simulink model "mcb_pmsm_foc_sensorless_f28069MLaunchPad"  (R2024a)
settings: Solver=FixedStepDiscrete  StartTime=0.0  StopTime=8  RelTol=1e-3  EnableMultiTasking=on
InitFcn:
  | mcb_pmsm_foc_sensorless_f28069MLaunchPad_datascript;
undefined symbols (not defined in the file): acceleration, Down, GPTRIP1SEL, GPTRIP2SEL, inverter, MAX_OL_NEG_SPD, MAX_OL_POS_SPD, MAX_OL_VD_LIMIT, MIN_CL_NEG_SPD, MIN_CL_POS_SPD, MIN_OL_VD_LIMIT, one_sec_tick, PI_params, pmsm, PU_System, RAMP_STEP_SIZE, target, Ts, Ts_motor, Ts_simulink, Ts_speed, two_sec_tick, TZ1, TZ2, Up
libraries: mcbcontrolslib x16, c2802xlib x5, simulink x4, c280xlib x4, slpidlib x3, mcbpositiondecoderlib x3, c2806xlib x3, mcbsensorlessestimatorlib x2, svdschedulerlib x2, mcbplantlib x1, autolibpmsmexterior x1
(part 1 of 3)
settings Model: ExtModeTrigDuration=8  Creator=The MathWorks, Inc.  LastModifiedBy=hirah
settings SolverCC: AlgebraicLoopSolver=TrustRegion  AutoInsertRateTranBlk=on
settings DataIOCC: LimitDataPoints=on  SaveFormat=Array  SaveOutput=off  SaveTime=off  ReturnWorkspaceOutputs=off
settings OptimizationCC: DefaultParameterBehavior=Inlined  DefaultUnderspecifiedDataType=single  OptimizeBlockIOStorage=off  BufferReuse=off  GlobalBufferReuse=off  ExpressionFolding=off  ExpressionDepthLimit=2147483647  LocalBlockOutputs=off  InitFltsAndDblsToZero=on  NoFixptDivByZeroProtection=on  EfficientFloat2IntCast=on  EfficientMapNaN2IntZero=off  LifeSpan=inf  MaxStackSize=1024  OptimizeDataStoreBuffers=off  BusAssignmentInplaceUpdate=off  DenormalBehavior=FlushToZero  EfficientTunableParamExpr=on
settings DebuggingCC: AlgebraicLoopMsg=error  ArtificialAlgebraicLoopMsg=error  CheckSSInitialOutputMsg=off  MergeDetectMultiDrivingBlocksExec=none  SolverPrmCheckMsg=warning  InheritedTsInSrcMsg=none  MultiTaskDSMMsg=none  MultiTaskCondExecSysMsg=none  TasksWithSamePriorityMsg=none  SigSpecEnsureSampleTimeMsg=none  ParameterPrecisionLossMsg=none  ParameterTunabilityLossMsg=error  FcnCallInpInsideContextMsg=warning  UnconnectedInputMsg=warning  UnconnectedOutputMsg=warning  UnconnectedLineMsg=warning  AllowSymbolicDim=off  StateNameClashWarn=warning  SFUnexpectedBacktrackingDiag=warning  SFNoUnconditionalDefaultTransitionDiag=warning  SFExecutionAtInitializationDiag=none  ArithmeticOperatorsInVariantConditions=warning
settings HardwareCC: ProdBitPerChar=16  ProdBitPerInt=16  ProdBitPerPointer=32  ProdBitPerSizeT=32  ProdBitPerPtrDiffT=32  ProdLargestAtomicInteger=Integer  ProdLargestAtomicFloat=None  ProdWordSize=16  ProdLongLongMode=on  ProdHWDeviceType=Texas Instruments->C2000  TargetBitPerChar=16  TargetBitPerInt=16  TargetBitPerPointer=16  TargetLargestAtomicInteger=Integer  TargetIntDivRoundTo=Zero  TargetEndianess=LittleEndian  TargetWordSize=16  TargetHWDeviceType=Texas Instruments->C2000
settings ModelReferenceCC: EnableRefExpFcnMdlSchedulingChecks=on  PropagateSignalLabelsOutOfModel=off
settings SFSimCC: SimUseLocalCustomCode=off  MATLABDynamicMemAlloc=off
settings RTWCC: Description=Embedded Coder  SystemTargetFile=ert.tlc  HardwareBoard=TI Piccolo F28069M LaunchPad  TemplateMakefile=ert_default_tmf  PostCodeGenCommand=; codertarget.postCodeGenHookCommand(h)  GenerateReport=on  RTWUseLocalCustomCode=off  Toolchain=Texas Instruments Code Composer Studio (C2000)  BuildConfiguration=Faster Runs  IncludeHyperlinkInReport=on  LaunchReport=on  GenerateTraceInfo=on  GenerateTraceReport=on  GenerateTraceReportSl=on  GenerateTraceReportSf=on  GenerateTraceReportEml=on  GPUComputeCapability=3.5  DLArmComputeVersion=19.05
settings CodeAppCC: IgnoreCustomStorageClasses=off  CustomSymbolStrType=$N$R$M  StateflowObjectComments=on  InternalIdentifier=Classic
settings ERTTargetCC: TargetFcnLib=ansi_tfl_tmw_new.mat  CodeReplacementLibrary=TI C28x  MultiwordLength=2048  ParMdlRefBuildCompliant=off  CompOptLevelCompliant=off  ConcurrentExecutionCompliant=off  CPPClassGenCompliant=off  ExtModeStaticAllocSize=2000  ExtModeMexFile=TIC2000ExternalModeOpen  ExtModeIntrfLevel=Level2 - Open  ConvertIfToSwitch=off  SuppressUnreachableDefaultCases=off  MemSecPackage=tic2000demospkg
settings ConfigComp: CovMetricSettings=dw  CovSaveCumulativeToWorkspaceVar=on  CovSaveSingleToWorkspaceVar=on  CovExternalEMLEnable=off  CovSFcnEnable=off

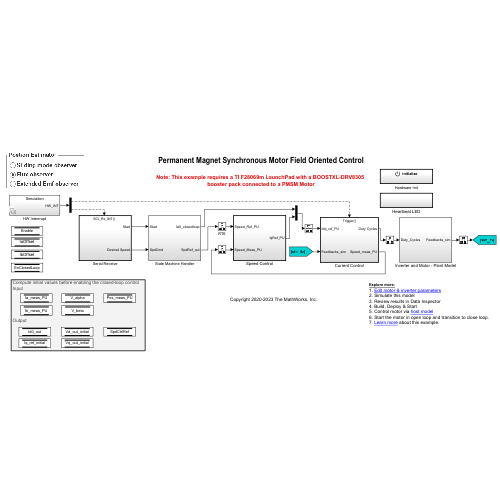
[thumbnail: Simulink's stored preview of the top-level diagram]
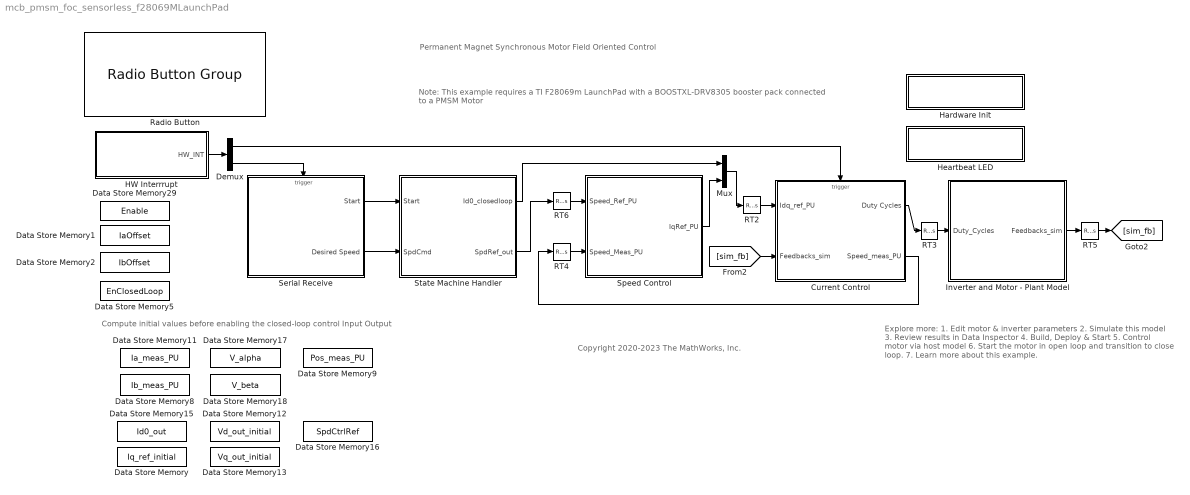
== system mcb_pmsm_foc_sensorless_f28069MLaunchPad ==
  note: Permanent Magnet Synchronous Motor Field Oriented Control
  note: Copyright 2020-2023 The MathWorks, Inc.
  note: Note: This example requires a TI F28069m LaunchPad with a BOOSTXL-DRV8305
      | booster pack connected to a PMSM Motor
  note: Explore more:
      | 1. Edit motor & inverter parameters
      | 2. Simulate this model
      | 3. Review results in Data Inspector
      | 4. Build, Deploy & Start
      | 5. Control motor via host model
      | 6. Start the motor in open loop and transition to close loop.
      | 7. Learn more about this example.
  note: Compute initial values before enabling the closed-loop control
      | Input
      |
      |
      |
      |
      |
      | Output
  Current Control : Subsystem
      settings: RTWSystemCode=Nonreusable function
  Data Store Memory : DataStoreMemory  DataStoreName=Iq_ref_initial  WriteAfterWriteMsg=warning  ShowAdditionalParam=off  OutDataTypeStr=dataType
  Data Store Memory1 : DataStoreMemory  DataStoreName=IaOffset  InitialValue=inverter.CtSensAOffset  ShowAdditionalParam=off
  Data Store Memory11 : DataStoreMemory  DataStoreName=Ia_meas_PU  WriteAfterWriteMsg=warning  ShowAdditionalParam=off  OutDataTypeStr=dataType
  Data Store Memory12 : DataStoreMemory  DataStoreName=Vd_out_initial  WriteAfterWriteMsg=warning  ShowAdditionalParam=off  OutDataTypeStr=dataType
  Data Store Memory13 : DataStoreMemory  DataStoreName=Vq_out_initial  WriteAfterWriteMsg=warning  ShowAdditionalParam=off  OutDataTypeStr=dataType
  Data Store Memory15 : DataStoreMemory  DataStoreName=Id0_out  InitialValue=0.1  ShowAdditionalParam=off  OutDataTypeStr=dataType
  Data Store Memory16 : DataStoreMemory  DataStoreName=SpdCtrlRef  InitialValue=0.1  ShowAdditionalParam=off  OutDataTypeStr=dataType
  Data Store Memory17 : DataStoreMemory  DataStoreName=V_alpha  WriteAfterWriteMsg=warning  ShowAdditionalParam=off  OutDataTypeStr=dataType
  Data Store Memory18 : DataStoreMemory  DataStoreName=V_beta  WriteAfterWriteMsg=warning  ShowAdditionalParam=off  OutDataTypeStr=dataType
  Data Store Memory2 : DataStoreMemory  DataStoreName=IbOffset  InitialValue=inverter.CtSensBOffset  ShowAdditionalParam=off
  Data Store Memory29 : DataStoreMemory  DataStoreName=Enable  ShowAdditionalParam=off  OutDataTypeStr=boolean
  Data Store Memory5 : DataStoreMemory  DataStoreName=EnClosedLoop  ReadBeforeWriteMsg=warning  WriteAfterWriteMsg=warning  WriteAfterReadMsg=warning  ShowAdditionalParam=off  OutDataTypeStr=boolean
  Data Store Memory8 : DataStoreMemory  DataStoreName=Ib_meas_PU  WriteAfterWriteMsg=warning  ShowAdditionalParam=off  OutDataTypeStr=dataType
  Data Store Memory9 : DataStoreMemory  DataStoreName=Pos_meas_PU  ShowAdditionalParam=off  OutDataTypeStr=dataType
  Demux : Demux  Outputs=2
  HW Interrrupt : Subsystem  Variant=on  VariantControlMode=sim codegen switching
  Hardware Init : Subsystem  TreatAsAtomicUnit=on
  Heartbeat LED : Subsystem  TreatAsAtomicUnit=on
  Inverter and Motor - Plant Model : Subsystem
  Mux : Mux  Inputs=2
  RT2 : RateTransition  Deterministic=off
  RT3 : RateTransition  Deterministic=off
  RT4 : RateTransition  Deterministic=off  OutPortSampleTime=Ts_speed
  RT5 : RateTransition  Deterministic=off
  RT6 : RateTransition  Deterministic=off  OutPortSampleTime=Ts_speed
  Radio Button : RadioButtonGroup  LabelPosition=Hide  SelectedLabel=Flux observer  ButtonGroupName=Postion Estimator
      settings: Values={{'Sliding mode observer', 'Flux observer', 'Extended Emf observer'}, [0 1 2]}
  Serial Receive : Subsystem  SystemSampleTime=1e-3
  Speed Control : Subsystem  Priority=50  TreatAsAtomicUnit=on  SystemSampleTime=Ts_speed
  State Machine Handler : Subsystem
  wires:
  Current Control/2(Speed_meas_PU) -> RT4/1
  Current Control/1(Duty Cycles) -> RT3/1
  HW Interrrupt/1(HW_INT) -> Demux/1
  RT3/1 -> Inverter and Motor - Plant Model/1(Duty_Cycles)
  RT2/1 -> Current Control/1(Idq_ref_PU)
  RT4/1 -> Speed Control/2(Speed_Meas_PU)
  Demux/1 -> Current Control/Trigger
  RT6/1 -> Speed Control/1(Speed_Ref_PU)
  Demux/2 -> Serial Receive/Trigger
  Inverter and Motor - Plant Model/1(Feedbacks_sim) -> RT5/1
  [sim_fb] -> Current Control/2(Feedbacks_sim)
  RT5/1 -> [sim_fb]
  State Machine Handler/2(SpdRef_out) -> RT6/1
  Speed Control/1(IqRef_PU) -> Mux/2
  Mux/1 -> RT2/1
  State Machine Handler/1(Id0_closedloop) -> Mux/1
  Serial Receive/1(Start) -> State Machine Handler/1(Start)
  Serial Receive/2(Desired Speed) -> State Machine Handler/2(SpdCmd)

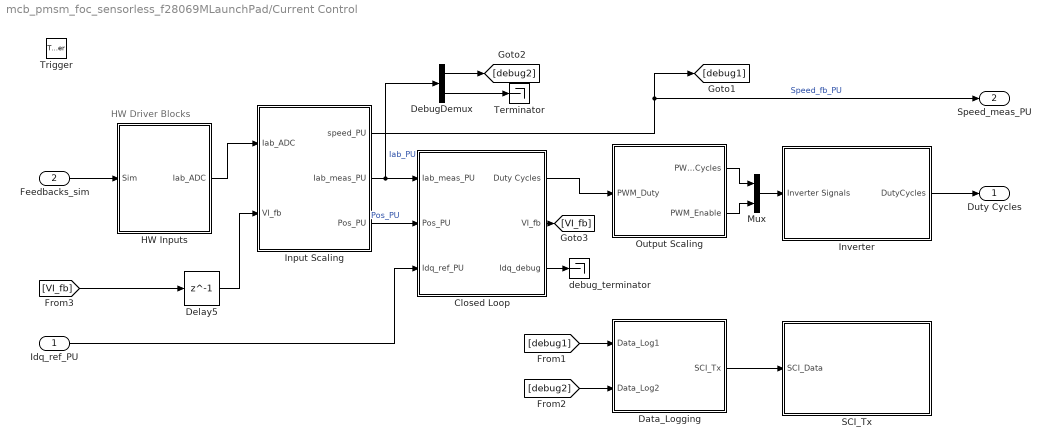
== system mcb_pmsm_foc_sensorless_f28069MLaunchPad/Current Control ==
  note: HW Driver Blocks
  Idq_ref_PU : Inport
  Feedbacks_sim : Inport  Port=2
  Trigger : TriggerPort  TriggerType=function-call  VariantControl=Variant  PortDimensions=1
  Closed Loop : Subsystem
  Data_Logging : Subsystem
  DebugDemux : Demux  Outputs=2
  Delay5 : Delay  DelayLength=1
  HW Inputs : Subsystem  Variant=on  VariantControlMode=sim codegen switching
  Input Scaling : Subsystem
  Inverter : Subsystem  Variant=on  VariantControlMode=sim codegen switching
  Mux : Mux  Inputs=2
  Output Scaling : Subsystem
  SCI_Tx : Subsystem  Variant=on  VariantControlMode=sim codegen switching
  Terminator : Terminator
  debug_terminator : Terminator
  Duty Cycles : Outport  InitialOutput=0  VectorParamsAs1DForOutWhenUnconnected=off
  Speed_meas_PU : Outport  Port=2  InitialOutput=0  VectorParamsAs1DForOutWhenUnconnected=off
  wires:
  Closed Loop/1(Duty Cycles) -> Output Scaling/1(PWM_Duty)
  Idq_ref_PU/1 -> Closed Loop/3(Idq_ref_PU)
  Output Scaling/2(PWM_Enable) -> Mux/2
  Input Scaling/1(speed_PU) -> Speed_meas_PU/1, [debug1]  "Speed_fb_PU"
  Feedbacks_sim/1 -> HW Inputs/1(Sim)
  Input Scaling/2(Iab_meas_PU) -> Closed Loop/1(Iab_meas_PU), DebugDemux/1  "Iab_PU"
  Input Scaling/3(Pos_PU) -> Closed Loop/2(Pos_PU)  "Pos_PU"
  [debug1] -> Data_Logging/1(Data_Log1)
  [debug2] -> Data_Logging/2(Data_Log2)
  Inverter/1(DutyCycles) -> Duty Cycles/1
  Output Scaling/1(PWM_Duty_Cycles) -> Mux/1
  Mux/1 -> Inverter/1(Inverter Signals)
  HW Inputs/1(Iab_ADC) -> Input Scaling/1(Iab_ADC)
  [VI_fb] -> Delay5/1
  Delay5/1 -> Input Scaling/2(VI_fb)
  Closed Loop/2(VI_fb) -> [VI_fb]
  DebugDemux/1 -> [debug2]
  DebugDemux/2 -> Terminator/1
  Closed Loop/3(Idq_debug) -> debug_terminator/1
  Data_Logging/1(SCI_Tx) -> SCI_Tx/1(SCI_Data)

== system mcb_pmsm_foc_sensorless_f28069MLaunchPad/HW Interrrupt ==
  Code generation : Subsystem  VariantControl=(codegen)
  Simulation : Subsystem  VariantControl=(sim)
  HW_INT : Outport  OutputFunctionCall=on

== system mcb_pmsm_foc_sensorless_f28069MLaunchPad/Hardware Init ==
  6PWM_Mode : Constant  Priority=1000  Value=0x3A16  OutDataTypeStr=uint16  SampleTime=-1
  ADC_Gain_Setting : Constant  Priority=1000  Value=inverter.SPI_Gain_Setting  OutDataTypeStr=uint16  SampleTime=-1
  Event Listener : EventListener  DisableCoverage=on  EventName=reset
  Mux : Mux  Inputs=2
  Variant Subsystem : Subsystem  Variant=on  VariantControlMode=sim codegen switching
  wires:
  6PWM_Mode/1 -> Mux/1
  ADC_Gain_Setting/1 -> Mux/2
  Mux/1 -> Variant Subsystem/1(In1)

== system mcb_pmsm_foc_sensorless_f28069MLaunchPad/Heartbeat LED ==
  note: Heartbeat LED 1HZ
  Heartbeat LED : Subsystem  Variant=on  VariantControlMode=sim codegen switching
  RED_LED : Constant  OutDataTypeStr=uint16  SampleTime=0.5
  wires:
  RED_LED/1 -> Heartbeat LED/1(In1)

== system mcb_pmsm_foc_sensorless_f28069MLaunchPad/Inverter and Motor - Plant Model ==
  Duty_Cycles : Inport
  Codegeneration : Subsystem
  Simulation : Subsystem
  Variant Sink : VariantSink  VariantControlMode=sim codegen switching
  Variant Source1 : VariantSource  VariantControlMode=sim codegen switching
  Feedbacks_sim : Outport  VectorParamsAs1DForOutWhenUnconnected=off
  wires:
  Duty_Cycles/1 -> Variant Sink/1
  Simulation/1(Feedbacks) -> Variant Source1/2
  Variant Sink/2 -> Simulation/1(Duty_Cycles)
  Variant Source1/1 -> Feedbacks_sim/1
  Variant Sink/1 -> Codegeneration/1(Duty_Cycles)
  Codegeneration/1(Feedbacks) -> Variant Source1/1

== system mcb_pmsm_foc_sensorless_f28069MLaunchPad/Serial Receive ==
  SCI_Rx_INT : TriggerPort  TriggerType=function-call  VariantControl=Variant
  Data Type Conversion1 : DataTypeConversion  OutDataTypeStr=dataType  RndMeth=Simplest  SaturateOnIntegerOverflow=off
  Data Type Conversion3 : DataTypeConversion  OutDataTypeStr=boolean  RndMeth=Simplest  SaturateOnIntegerOverflow=off
  Data_Conditioning : Subsystem
  Demux : Demux  Outputs=2
  SCI_Rx : Subsystem  Variant=on  VariantControlMode=sim codegen switching
  Start : Outport  VectorParamsAs1DForOutWhenUnconnected=off
  Desired Speed : Outport  Port=2  VectorParamsAs1DForOutWhenUnconnected=off
  wires:
  Data Type Conversion1/1 -> Desired Speed/1  "Speed_Ref"
  Demux/1 -> Data Type Conversion1/1
  Data_Conditioning/1(Out1) -> Demux/1
  Data Type Conversion3/1 -> Start/1
  Demux/2 -> Data Type Conversion3/1
  SCI_Rx/1(Data) -> Data_Conditioning/1(Data)

== system mcb_pmsm_foc_sensorless_f28069MLaunchPad/Speed Control ==
  Speed_Ref_PU : Inport
  Speed_Meas_PU : Inport  Port=2
  PI_Controller_Speed : Subsystem
  SlewRate : Subsystem
  IqRef_PU : Outport  VectorParamsAs1DForOutWhenUnconnected=off
  wires:
  Speed_Meas_PU/1 -> PI_Controller_Speed/2(N_fb)  "Speed_fb"
  Speed_Ref_PU/1 -> SlewRate/1(Speed_Ref)
  SlewRate/1(N_ref) -> PI_Controller_Speed/1(N_ref)  "Speed_ref"
  PI_Controller_Speed/1(Iq_ref) -> IqRef_PU/1

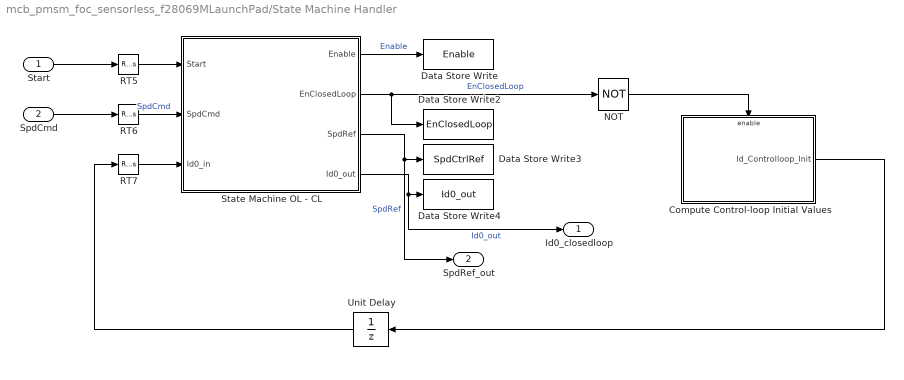
== system mcb_pmsm_foc_sensorless_f28069MLaunchPad/State Machine Handler ==
  Start : Inport
  SpdCmd : Inport  Port=2
  Compute Control-loop Initial Values : Subsystem
  Data Store Write : DataStoreWrite  DataStoreName=Enable  IndexOptions=Index vector (dialog)  Indices=1  OutputSizes=1
  Data Store Write2 : DataStoreWrite  DataStoreName=EnClosedLoop  IndexOptions=Index vector (dialog)  Indices=1  OutputSizes=1
  Data Store Write3 : DataStoreWrite  DataStoreName=SpdCtrlRef  IndexOptions=Index vector (dialog)  Indices=1  OutputSizes=1
  Data Store Write4 : DataStoreWrite  DataStoreName=Id0_out  IndexOptions=Index vector (dialog)  Indices=1  OutputSizes=1
  NOT : Logic  Operator=NOT  IconShape=distinctive  AllPortsSameDT=off  OutDataTypeStr=boolean
  RT5 : RateTransition  Deterministic=off  OutPortSampleTime=Ts_speed
  RT6 : RateTransition  Deterministic=off  OutPortSampleTime=Ts_speed
  RT7 : RateTransition  Deterministic=off  OutPortSampleTime=Ts_speed
  State Machine OL - CL : Stateflow chart  Priority=10  TreatAsAtomicUnit=on  SystemSampleTime=Ts_speed
  Unit Delay : UnitDelay  SampleTime=-1  HasFrameUpgradeWarning=on
  Id0_closedloop : Outport
  SpdRef_out : Outport  Port=2
  wires:
  State Machine OL - CL/4(Id0_out) -> Id0_closedloop/1, Data Store Write4/1  "Id0_out"
  State Machine OL - CL/2(EnClosedLoop) -> Data Store Write2/1, NOT/1  "EnClosedLoop"
  RT6/1 -> State Machine OL - CL/2(SpdCmd)  "SpdCmd"
  Start/1 -> RT5/1
  State Machine OL - CL/3(SpdRef) -> SpdRef_out/1, Data Store Write3/1  "SpdRef"
  RT5/1 -> State Machine OL - CL/1(Start)
  State Machine OL - CL/1(Enable) -> Data Store Write/1  "Enable"
  SpdCmd/1 -> RT6/1
  Compute Control-loop Initial Values/1(Id_Controlloop_Init) -> Unit Delay/1
  Unit Delay/1 -> RT7/1
  NOT/1 -> Compute Control-loop Initial Values/Enable
  RT7/1 -> State Machine OL - CL/3(Id0_in)

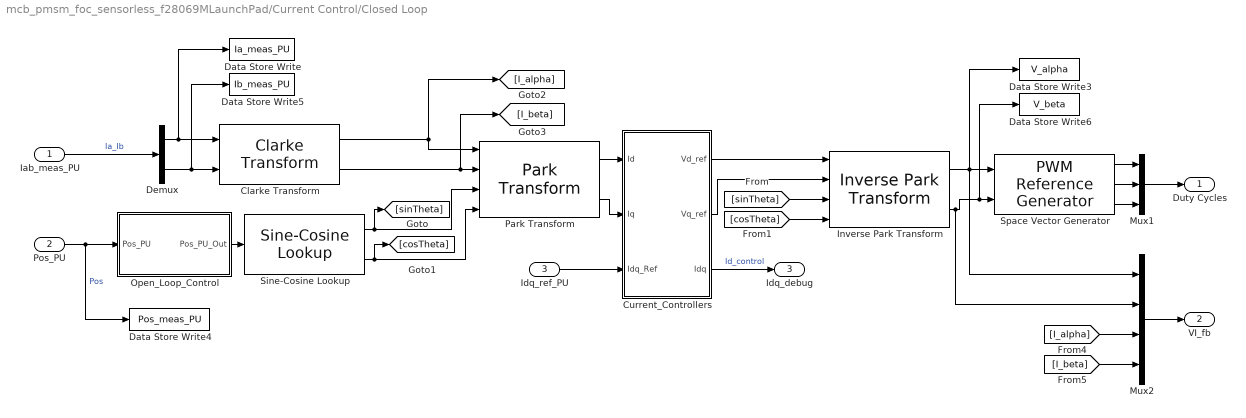
== system mcb_pmsm_foc_sensorless_f28069MLaunchPad/Current Control/Closed Loop ==
  Iab_meas_PU : Inport
  Pos_PU : Inport  Port=2
  Idq_ref_PU : Inport  Port=3
  Clarke Transform : mcbcontrolslib/Clarke Transform  VariantControl=Variant2  PhaseInput=Two inputs  EnPowerInv=off
  Current_Controllers : Subsystem
  Data Store Write : DataStoreWrite  DataStoreName=Ia_meas_PU  IndexOptions=Index vector (dialog)  Indices=1  OutputSizes=1
  Data Store Write3 : DataStoreWrite  DataStoreName=V_alpha  IndexOptions=Index vector (dialog)  Indices=1  OutputSizes=1
  Data Store Write4 : DataStoreWrite  DataStoreName=Pos_meas_PU  IndexOptions=Index vector (dialog)  Indices=1  OutputSizes=1
  Data Store Write5 : DataStoreWrite  DataStoreName=Ib_meas_PU  IndexOptions=Index vector (dialog)  Indices=1  OutputSizes=1
  Data Store Write6 : DataStoreWrite  DataStoreName=V_beta  IndexOptions=Index vector (dialog)  Indices=1  OutputSizes=1
  Demux : Demux  Outputs=2
  Inverse Park Transform : mcbcontrolslib/Inverse Park Transform  PhaseInput=Two inputs  AxisAlignment=D-axis  ThetaInput=Sine and Cosine electrical position  AngleInput=Per-unit  N_points=1024
  Mux1 : Mux  Inputs=3
  Mux2 : Mux
  Open_Loop_Control : Subsystem
  Park Transform : mcbcontrolslib/Park Transform  PhaseInput=Two inputs  AxisAlignment=D-axis  ThetaInput=Sine and Cosine electrical position  AngleInput=Per-unit  N_points=1024
  Sine-Cosine Lookup : mcbcontrolslib/Sine-Cosine Lookup  AngleInput=Per-unit  N_points=1024  DatatypeInput=Inherit from input  Datatype=single
  Space Vector Generator : mcbcontrolslib/PWM Reference Generator  inSignal=Valphabeta  modType=SVM: space vector modulation
  Duty Cycles : Outport  VectorParamsAs1DForOutWhenUnconnected=off
  VI_fb : Outport  Port=2  VectorParamsAs1DForOutWhenUnconnected=off
  Idq_debug : Outport  Port=3  VectorParamsAs1DForOutWhenUnconnected=off
  wires:
  Current_Controllers/1(Vd_ref) -> Inverse Park Transform/1
  [cosTheta] -> Inverse Park Transform/4
  [I_beta] -> Mux2/4
  Inverse Park Transform/2 -> Mux2/2, Data Store Write6/1, Space Vector Generator/2
  Inverse Park Transform/1 -> Data Store Write3/1, Mux2/1, Space Vector Generator/1
  [sinTheta] -> Inverse Park Transform/3
  Mux2/1 -> VI_fb/1
  Clarke Transform/1 -> Park Transform/1, [I_alpha]
  Current_Controllers/2(Vq_ref) -> Inverse Park Transform/2
  Clarke Transform/2 -> [I_beta], Park Transform/2
  Sine-Cosine Lookup/1 -> [sinTheta], Park Transform/3
  [I_alpha] -> Mux2/3
  Space Vector Generator/1 -> Mux1/1
  Space Vector Generator/3 -> Mux1/3
  Mux1/1 -> Duty Cycles/1
  Sine-Cosine Lookup/2 -> Park Transform/4, [cosTheta]
  Space Vector Generator/2 -> Mux1/2
  Park Transform/1 -> Current_Controllers/1(Id)
  Park Transform/2 -> Current_Controllers/2(Iq)
  Demux/1 -> Data Store Write/1, Clarke Transform/1
  Demux/2 -> Data Store Write5/1, Clarke Transform/2
  Iab_meas_PU/1 -> Demux/1  "Ia_Ib"
  Idq_ref_PU/1 -> Current_Controllers/3(Idq_Ref)
  Pos_PU/1 -> Data Store Write4/1, Open_Loop_Control/1(Pos_PU)  "Pos"
  Current_Controllers/3(Idq) -> Idq_debug/1  "Id_control"
  Open_Loop_Control/1(Pos_PU_Out) -> Sine-Cosine Lookup/1

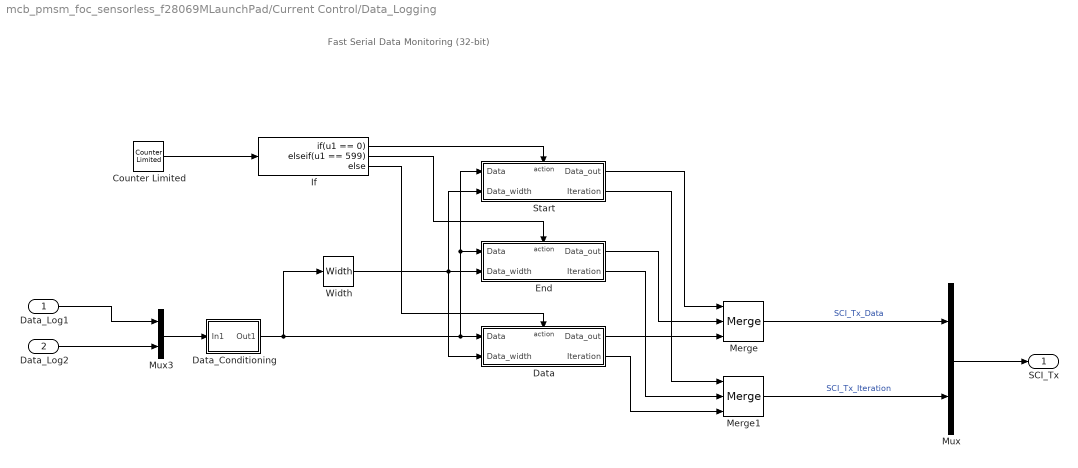
== system mcb_pmsm_foc_sensorless_f28069MLaunchPad/Current Control/Data_Logging ==
  note: Fast Serial Data Monitoring (32-bit)
  Data_Log1 : Inport
  Data_Log2 : Inport  Port=2
  Counter Limited : simulink/Sources/Counter Limited  uplimit=599  tsamp=-1
  Data : Subsystem  TreatAsAtomicUnit=on
  Data_Conditioning : Subsystem
  End : Subsystem  TreatAsAtomicUnit=on
  If : If  IfExpression=u1 == 0  ElseIfExpressions=u1 == 599
  Merge : Merge  Inputs=3
  Merge1 : Merge  Inputs=3
  Mux : Mux  Inputs=2
  Mux3 : Mux  Inputs=2
  Start : Subsystem  TreatAsAtomicUnit=on
  Width : Width  OutDataTypeMode=All ports same datatype  DataType=uint16
  SCI_Tx : Outport
  wires:
  If/3 -> Data/Action
  Data/1(Data_out) -> Merge/3
  Width/1 -> Data/2(Data_width), Start/2(Data_width), End/2(Data_width)
  Merge/1 -> Mux/1  "SCI_Tx_Data"
  Counter Limited/1 -> If/1
  Start/2(Iteration) -> Merge1/1
  Start/1(Data_out) -> Merge/1
  If/2 -> End/Action
  Merge1/1 -> Mux/2  "SCI_Tx_Iteration"
  If/1 -> Start/Action
  End/1(Data_out) -> Merge/2
  End/2(Iteration) -> Merge1/2
  Data/2(Iteration) -> Merge1/3
  Data_Log1/1 -> Mux3/1
  Data_Conditioning/1(Out1) -> Width/1, Start/1(Data), End/1(Data), Data/1(Data)
  Mux/1 -> SCI_Tx/1
  Mux3/1 -> Data_Conditioning/1(In1)
  Data_Log2/1 -> Mux3/2

== system mcb_pmsm_foc_sensorless_f28069MLaunchPad/Current Control/HW Inputs ==
  Sim : Inport
  Sensor Driver Blocks (codegen) : Subsystem  VariantControl=(codegen)
  Sensor Driver Blocks (sim) : Subsystem  VariantControl=(sim)
  Iab_ADC : Outport

== system mcb_pmsm_foc_sensorless_f28069MLaunchPad/Current Control/Input Scaling ==
  note: Current Measurements
  Iab_ADC : Inport
  VI_fb : Inport  Port=2
  Calculate Phase Currents : Subsystem
  Calculate position and speed : Subsystem
  speed_PU : Outport
  Iab_meas_PU : Outport  Port=2
  Pos_PU : Outport  Port=3
  wires:
  Calculate Phase Currents/1(Iab_meas_PU) -> Iab_meas_PU/1  "Iab_fb_PU"
  Iab_ADC/1 -> Calculate Phase Currents/1(Iab_ADC)
  Calculate position and speed/2(speed_PU) -> speed_PU/1
  Calculate position and speed/1(Pos_PU) -> Pos_PU/1
  VI_fb/1 -> Calculate position and speed/1(VI_fb)

== system mcb_pmsm_foc_sensorless_f28069MLaunchPad/Current Control/Inverter ==
  Inverter Signals : Inport
  Code Generation : Subsystem  VariantControl=(codegen)
  Simulation : Subsystem  VariantControl=(sim)
  DutyCycles : Outport  VectorParamsAs1DForOutWhenUnconnected=off

== system mcb_pmsm_foc_sensorless_f28069MLaunchPad/Current Control/Output Scaling ==
  PWM_Duty : Inport
  Constant : Constant  Value=0.5  OutDataTypeStr=dataType
  Data Type Conversion : DataTypeConversion  OutDataTypeStr=dataType  SaturateOnIntegerOverflow=off  RndMeth=Floor
  Enable : DataStoreRead  DataStoreName=Enable  IndexOptions=Index vector (dialog)  Indices=1  OutputSizes=1
  Gain : Gain  Gain=0.5  OutDataTypeStr=Inherit: Same as input
  Sum : Sum  Inputs=|++
  PWM_Duty_Cycles : Outport
  PWM_Enable : Outport  Port=2
  wires:
  Sum/1 -> PWM_Duty_Cycles/1  "PWM_Duty_Cycles"
  Constant/1 -> Sum/2
  Gain/1 -> Sum/1
  PWM_Duty/1 -> Gain/1
  Data Type Conversion/1 -> PWM_Enable/1
  Enable/1 -> Data Type Conversion/1

== system mcb_pmsm_foc_sensorless_f28069MLaunchPad/Current Control/SCI_Tx ==
  SCI_Data : Inport
  Code Generation : Subsystem  VariantControl=(codegen)
  Simulation : Subsystem  VariantControl=(sim)

== system mcb_pmsm_foc_sensorless_f28069MLaunchPad/HW Interrrupt/Code generation ==
  HWI_ADCINT1 : svdschedulerlib/Hardware Interrupt v2  ISRGroup=ADC - Analog to Digital Converter  ISRName=ADCA1_INT  ISRNumber=32  NumEventsToServe=1  EventsList={'on','EOC event','1';'off','Overflow event','2';'off','Custom event','3'}  SelectedEvents={'event1'}  TaskPriority=30  DisablePreemption=on  ClearInterruptFlagsAtEndOfEvent=on  InterruptDefinitionFile=$(TARGET_ROOT)/registry/interrupts/F2837xS_interrupts.xml  HardwareBoard=F2837x  EnableSimPort=off
      settings: LibrarySourceBlock=c2000lib/Scheduling/Hardware Interrupt
  HWI_SCIRXINTA : svdschedulerlib/Hardware Interrupt v2  ISRGroup=ADC - Analog to Digital Converter  ISRName=ADCA1_INT  ISRNumber=32  NumEventsToServe=1  EventsList={'on','EOC event','1';'off','Overflow event','2';'off','Custom event','3'}  SelectedEvents={'event1'}  TaskPriority=25  DisablePreemption=off  ClearInterruptFlagsAtEndOfEvent=on  InterruptDefinitionFile=$(TARGET_ROOT)/registry/interrupts/F2837xS_interrupts.xml  HardwareBoard=F2837x  EnableSimPort=off
      settings: LibrarySourceBlock=c2000lib/Scheduling/Hardware Interrupt
  Mux : Mux  Inputs=2
  HW_INT : Outport
  wires:
  Mux/1 -> HW_INT/1
  HWI_ADCINT1/1 -> Mux/1
  HWI_SCIRXINTA/1 -> Mux/2

== system mcb_pmsm_foc_sensorless_f28069MLaunchPad/HW Interrrupt/Simulation ==
  ADCINT1 : simulink/Ports & Subsystems/Function-Call Generator  sample_time=Ts  numberOfIterations=1  DisallowWideOutput=off
  Mux : Mux  Inputs=2
  SCI_Rx_INT : simulink/Ports & Subsystems/Function-Call Generator  sample_time=0.1  numberOfIterations=1  DisallowWideOutput=off
  HW_INT : Outport
  wires:
  SCI_Rx_INT/1 -> Mux/2
  ADCINT1/1 -> Mux/1
  Mux/1 -> HW_INT/1

== system mcb_pmsm_foc_sensorless_f28069MLaunchPad/Hardware Init/Variant Subsystem ==
  In1 : Inport
  Code Generation : Subsystem  VariantControl=(codegen)
  Simulation : Subsystem  VariantControl=(sim)

== system mcb_pmsm_foc_sensorless_f28069MLaunchPad/Heartbeat LED/Heartbeat LED ==
  In1 : Inport
  Code generation : Subsystem  VariantControl=(codegen)
  Simulation : Subsystem  VariantControl=(sim)

== system mcb_pmsm_foc_sensorless_f28069MLaunchPad/Inverter and Motor - Plant Model/Codegeneration ==
  Duty_Cycles : Inport
  Ground : Ground
  Terminator : Terminator
  Feedbacks : Outport  VectorParamsAs1DForOutWhenUnconnected=off
  wires:
  Duty_Cycles/1 -> Terminator/1
  Ground/1 -> Feedbacks/1

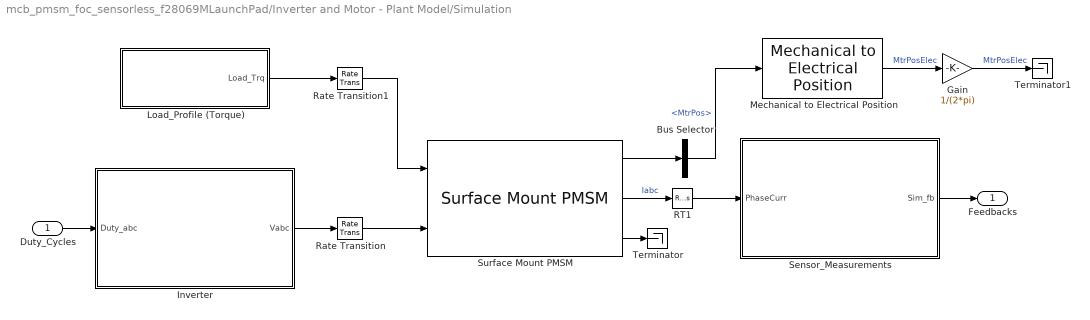
== system mcb_pmsm_foc_sensorless_f28069MLaunchPad/Inverter and Motor - Plant Model/Simulation ==
  Duty_Cycles : Inport
  Bus Selector : BusSelector  OutputSignals=MtrPos
  Gain : Gain  Gain=1/(2*pi)  OutDataTypeStr=Inherit: Same as input
  Inverter : Subsystem
  Load_Profile (Torque) : Subsystem
  Mechanical to Electrical Position : mcbpositiondecoderlib/Mechanical to Electrical Position  PolePairsInputType=Specify via dialog  NrPP=pmsm.p  selectedRange=Radians  MechOfstInputType=Specify via dialog  mechOffsetIn=0  maxAngleIn=2*pi  InputDataType=single  VariantSelect=floating-point
  RT1 : RateTransition  Deterministic=off  OutPortSampleTime=Ts_simulink
  Rate Transition : RateTransition  Deterministic=off  OutPortSampleTime=Ts_motor
  Rate Transition1 : RateTransition  Deterministic=off  OutPortSampleTime=Ts_motor
  Sensor_Measurements : Subsystem
  Surface Mount PMSM : autolibpmsmexterior/Surface Mount PMSM  port_config=Torque  sim_type=Discrete  Ts=Ts_motor  P=pmsm.p  Rs=pmsm.Rs + inverter.R_board  Ldq_=pmsm.Ld  KConstText=Permanent flux linkage constant (lambda_pm):  lambda_pm=pmsm.FluxPM  Ke=159.9771  Kt=1.323  mechanical=[pmsm.J, pmsm.B, 0]  idq0=[0 0]  theta_init=0  omega_init=0  KConst=pmsm.FluxPM  lambda_pm_calc=pmsm.FluxPM  RefBlkName='autolibpmsmexterior/Surface Mount PMSM'  aMode=5  Ldq="[0.0002      0.0002]"
  Terminator : Terminator
  Terminator1 : Terminator
  Feedbacks : Outport  VectorParamsAs1DForOutWhenUnconnected=off
  wires:
  RT1/1 -> Sensor_Measurements/1(PhaseCurr)
  Surface Mount PMSM/2 -> RT1/1  "Iabc"
  Sensor_Measurements/1(Sim_fb) -> Feedbacks/1
  Gain/1 -> Terminator1/1  "MtrPosElec"
  Inverter/1(Vabc) -> Rate Transition/1
  Surface Mount PMSM/3 -> Terminator/1
  Surface Mount PMSM/1 -> Bus Selector/1
  Mechanical to Electrical Position/1 -> Gain/1  "MtrPosElec"
  Duty_Cycles/1 -> Inverter/1(Duty_abc)
  Rate Transition/1 -> Surface Mount PMSM/2
  Bus Selector/1 -> Mechanical to Electrical Position/1  "<MtrPos>"
  Rate Transition1/1 -> Surface Mount PMSM/1
  Load_Profile (Torque)/1(Load_Trq) -> Rate Transition1/1

== system mcb_pmsm_foc_sensorless_f28069MLaunchPad/Serial Receive/Data_Conditioning ==
  Data : Inport
  Data Type Conversion1 : DataTypeConversion  OutDataTypeStr=single  RndMeth=Simplest  SaturateOnIntegerOverflow=off
  Data Type Conversion2 : DataTypeConversion  OutDataTypeStr=fixdt(1,16,12)  ConvertRealWorld=Stored Integer (SI)  RndMeth=Simplest  SaturateOnIntegerOverflow=off
  Out1 : Outport  VectorParamsAs1DForOutWhenUnconnected=off
  wires:
  Data Type Conversion1/1 -> Out1/1
  Data/1 -> Data Type Conversion2/1
  Data Type Conversion2/1 -> Data Type Conversion1/1

== system mcb_pmsm_foc_sensorless_f28069MLaunchPad/Serial Receive/SCI_Rx ==
  Code Generation : Subsystem  VariantControl=(codegen)
  Simulation : Subsystem  VariantControl=(sim)
  Data : Outport

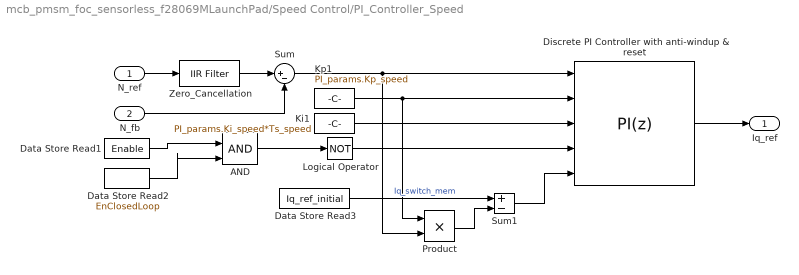
== system mcb_pmsm_foc_sensorless_f28069MLaunchPad/Speed Control/PI_Controller_Speed ==
  N_ref : Inport
  N_fb : Inport  Port=2
  AND : Logic  IconShape=distinctive  AllPortsSameDT=off  OutDataTypeStr=boolean
  Data Store Read2 : DataStoreRead  DataStoreName=EnClosedLoop  IndexOptions=Index vector (dialog)  Indices=1  OutputSizes=1
  Data Store Read3 : DataStoreRead  DataStoreName=Iq_ref_initial  IndexOptions=Index vector (dialog)  Indices=1  OutputSizes=1
  Data Store Read1 : DataStoreRead  DataStoreName=Enable  IndexOptions=Index vector (dialog)  Indices=1  OutputSizes=1
  Discrete PI Controller with anti-windup & reset : slpidlib/PID Controller  Controller=PI  Form=Parallel  TimeDomain=Discrete-time  UseExternalTs=off  SampleTime=-1  IntegratorMethod=Forward Euler  FilterMethod=Forward Euler  ControllerParametersSource=external  P=1  I=1  UseKiTs=on  D=0  UseExternalDerivativeSource=off  N=100  UseFilter=on  TunerSelectOption=Transfer Function Based (PID Tuner App)  InitialConditionSource=external  InitialConditionForIntegrator=0  InitialConditionForFilter=0  DifferentiatorICPrevScaledInput=0  ExternalReset=level  TrackingMode=off  Kt=1  LimitOutput=on  SatLimitsSource=internal  UpperSaturationLimit=1  LowerSaturationLimit=-1  LinearizeAsGain=on  AntiWindupMode=clamping  Kb=1  LimitIntegrator=off  UpperIntegratorSaturationLimit=inf  LowerIntegratorSaturationLimit=-inf  RndMeth=Simplest  POutMin=[]  POutMax=[]  IOutMin=[]  IOutMax=[]  DOutMin=[]  DOutMax=[]  NOutMin=[]  NOutMax=[]  SumOutMin=[]  SumOutMax=[]  SaturationOutDataTypeStr=Inherit: Inherit via back propagation  SaturationOutMin=[]  SaturationOutMax=[]  PParamMin=[]  PParamMax=[]  IParamMin=[]  IParamMax=[]  DParamMin=[]  DParamMax=[]  NParamMin=[]  NParamMax=[]  KbParamMin=[]  KbParamMax=[]  KtParamMin=[]  KtParamMax=[]  KbOutMin=[]  KbOutMax=[]  KtOutMin=[]  KtOutMax=[]  IntegratorOutMin=[]  IntegratorOutMax=[]  FilterOutMin=[]  FilterOutMax=[]  SumI1OutMin=[]  SumI1OutMax=[]  SumI2OutMin=[]  SumI2OutMax=[]  SumI3OutMin=[]  SumI3OutMax=[]  SumI4OutMin=[]  SumI4OutMax=[]  SumDOutMin=[]  SumDOutMax=[]  DifferentiatorOutMin=[]  DifferentiatorOutMax=[]  FilterDiffOutCoefMin=[]  FilterDiffOutCoefMax=[]  ReciprocalOutMin=[]  ReciprocalOutMax=[]  SumDenOutMin=[]  SumDenOutMax=[]  SumNumOutMin=[]  SumNumOutMax=[]  DivideOutMin=[]  DivideOutMax=[]  UdiffTsProdOutMin=[]  UdiffTsProdOutMax=[]  NTsProdOutMin=[]  NTsProdOutMax=[]  UintegralTsProdOutMin=[]  UintegralTsProdOutMax=[]  UngainTsProdOutMin=[]  UngainTsProdOutMax=[]  ClampingZeroOutDataTypeStr=Inherit: Inherit via back propagation  ClampingZeroOutMin=[]  ClampingZeroOutMax=[]  FilterDenConstantOutDataTypeStr=Inherit: Inherit via back propagation  FilterDenConstantOutMin=[]  FilterDenConstantOutMax=[]  PCopyOutDataTypeStr=Inherit: Inherit via back propagation  PCopyOutMin=[]  PCopyOutMax=[]  NCopyOutDataTypeStr=Inherit: Inherit via back propagation  NCopyOutMin=[]  NCopyOutMax=[]  IntegratorContinuousStateAttributes=''  IntegratorStateMustResolveToSignalObject=off  IntegratorRTWStateStorageClass=Auto  FilterContinuousStateAttributes=''  FilterStateMustResolveToSignalObject=off  FilterRTWStateStorageClass=Auto  ParallelPVariant=ExternalParameters  IdealPVariant=Disabled  IVariant=ExternalParameters  DVariant=Disabled  IntegratorVariant=Discrete  SatVariant=Enabled  AWVariant=DiscClampingParallel  PCopyVariant=Disabled  TRVariant=Disabled  FdbkBlocksVariant=Forward  IdealPFdbkVariant=Disabled  SatFdbkVariant=Disabled  DerivativeFilterVariant=Disabled  NVariant=Disabled  NCopyVariant=Disabled_SignalSpec  FilterICVariant=Disabled  IntegratorICVariant=ExternalICs  ExternalResetVariant=ExternalReset  TRSumVariant=Passthrough  SumFdbkVariant=Disabled  SumVariant=Sum_PI  TsampFilterVariant=InternalTs  TsampNgainVariant=Passthrough  TsampIntegralVariant=Disabled_SignalSpec  ExternalSaturationOutDataTypeStr=Inherit: Same as second input  DerivativeSourceVariant=Disabled
      settings: LibrarySourceBlock=mcbcontrolslib/PI Controller
  Ki1 : Constant  Value=PI_params.Ki_speed*Ts_speed  OutDataTypeStr=dataType  SampleTime=-1
  Kp1 : Constant  Value=PI_params.Kp_speed  OutDataTypeStr=dataType  SampleTime=-1
  Logical Operator : Logic  Operator=NOT  IconShape=distinctive  AllPortsSameDT=off  OutDataTypeStr=boolean
  Product : Product  OutDataTypeStr=Inherit: Same as first input
  Sum : Sum  Inputs=|+-  OutDataTypeStr=Inherit: Same as first input
  Sum1 : Sum  Inputs=+-  OutDataTypeStr=Inherit: Same as first input
  Zero_Cancellation : mcbcontrolslib/IIR Filter  VariantControl=Low Pass Filter  VariantSelect=Low-pass  FilterConstantInputType=Specify via dialog  Filter_constant=0.01*(Ts_speed/Ts)  advancedSettings=off  Ts=50e-6  cutOff_freq=1
  Iq_ref : Outport  VectorParamsAs1DForOutWhenUnconnected=off
  wires:
  Discrete PI Controller with anti-windup & reset/1 -> Iq_ref/1
  Ki1/1 -> Discrete PI Controller with anti-windup & reset/3
  Kp1/1 -> Product/1, Discrete PI Controller with anti-windup & reset/2
  N_fb/1 -> Sum/2
  N_ref/1 -> Zero_Cancellation/1
  Logical Operator/1 -> Discrete PI Controller with anti-windup & reset/4
  Sum1/1 -> Discrete PI Controller with anti-windup & reset/5
  Data Store Read1/1 -> AND/1
  Data Store Read2/1 -> AND/2
  AND/1 -> Logical Operator/1
  Zero_Cancellation/1 -> Sum/1
  Sum/1 -> Product/2, Discrete PI Controller with anti-windup & reset/1
  Product/1 -> Sum1/2
  Data Store Read3/1 -> Sum1/1  "Iq_switch_mem"

== system mcb_pmsm_foc_sensorless_f28069MLaunchPad/Speed Control/SlewRate ==
  Speed_Ref : Inport
  Rate Limiter : RateLimiter  RisingSlewLimit=acceleration  FallingSlewLimit=-acceleration  SampleTimeMode=inherited  InitialCondition=MAX_OL_POS_SPD
  Rate Limiter1 : RateLimiter  RisingSlewLimit=acceleration  FallingSlewLimit=-acceleration  SampleTimeMode=inherited  InitialCondition=MAX_OL_NEG_SPD
  Switch : Switch  SaturateOnIntegerOverflow=off  InputSameDT=off
  N_ref : Outport
  wires:
  Switch/1 -> N_ref/1
  Rate Limiter/1 -> Switch/1
  Rate Limiter1/1 -> Switch/3
  Speed_Ref/1 -> Rate Limiter/1, Rate Limiter1/1, Switch/2

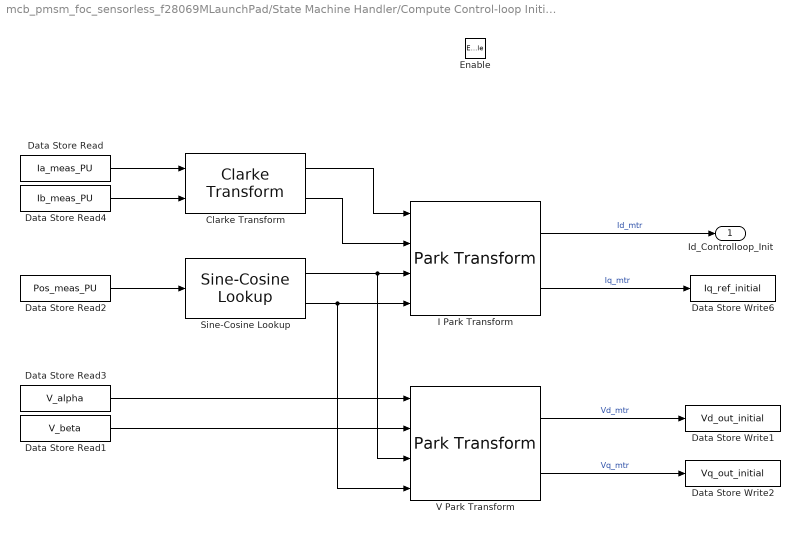
== system mcb_pmsm_foc_sensorless_f28069MLaunchPad/State Machine Handler/Compute Control-loop Initial Values ==
  Enable : EnablePort
  Clarke Transform : mcbcontrolslib/Clarke Transform  VariantControl=Variant2  PhaseInput=Two inputs  EnPowerInv=off
  Data Store Read : DataStoreRead  DataStoreName=Ia_meas_PU  IndexOptions=Index vector (dialog)  Indices=1  OutputSizes=1
  Data Store Read1 : DataStoreRead  DataStoreName=V_beta  IndexOptions=Index vector (dialog)  Indices=1  OutputSizes=1
  Data Store Read2 : DataStoreRead  DataStoreName=Pos_meas_PU  IndexOptions=Index vector (dialog)  Indices=1  OutputSizes=1
  Data Store Read3 : DataStoreRead  DataStoreName=V_alpha  IndexOptions=Index vector (dialog)  Indices=1  OutputSizes=1
  Data Store Read4 : DataStoreRead  DataStoreName=Ib_meas_PU  IndexOptions=Index vector (dialog)  Indices=1  OutputSizes=1
  Data Store Write1 : DataStoreWrite  DataStoreName=Vd_out_initial  IndexOptions=Index vector (dialog)  Indices=1  OutputSizes=1
  Data Store Write2 : DataStoreWrite  DataStoreName=Vq_out_initial  IndexOptions=Index vector (dialog)  Indices=1  OutputSizes=1
  Data Store Write6 : DataStoreWrite  DataStoreName=Iq_ref_initial  IndexOptions=Index vector (dialog)  Indices=1  OutputSizes=1
  I Park Transform : mcbcontrolslib/Park Transform  PhaseInput=Two inputs  AxisAlignment=D-axis  ThetaInput=Sine and Cosine electrical position  AngleInput=Per-unit  N_points=1024
  Sine-Cosine Lookup : mcbcontrolslib/Sine-Cosine Lookup  AngleInput=Per-unit  N_points=1024  DatatypeInput=Inherit from input  Datatype=single
  V Park Transform : mcbcontrolslib/Park Transform  PhaseInput=Two inputs  AxisAlignment=D-axis  ThetaInput=Sine and Cosine electrical position  AngleInput=Per-unit  N_points=1024
  Id_Controlloop_Init : Outport
  wires:
  Clarke Transform/1 -> I Park Transform/1
  Sine-Cosine Lookup/1 -> V Park Transform/3, I Park Transform/3
  I Park Transform/1 -> Id_Controlloop_Init/1  "Id_mtr"
  I Park Transform/2 -> Data Store Write6/1  "Iq_mtr"
  Clarke Transform/2 -> I Park Transform/2
  Data Store Read2/1 -> Sine-Cosine Lookup/1
  Sine-Cosine Lookup/2 -> V Park Transform/4, I Park Transform/4
  Data Store Read4/1 -> Clarke Transform/2
  Data Store Read3/1 -> V Park Transform/1
  Data Store Read1/1 -> V Park Transform/2
  V Park Transform/1 -> Data Store Write1/1  "Vd_mtr"
  V Park Transform/2 -> Data Store Write2/1  "Vq_mtr"
  Data Store Read/1 -> Clarke Transform/1

== system mcb_pmsm_foc_sensorless_f28069MLaunchPad/State Machine Handler/State Machine OL - CL/RunMode.ComputeId0 ==
  Id0_in : Inport  OutDataTypeStr=dataType  PortDimensions=1
  RAMP_STEP_SIZE : Inport  Port=2  OutDataTypeStr=dataType  PortDimensions=1
  f : TriggerPort  TriggerType=function-call  VariantControl=(inherit)
      settings: CopyFcn=Stateflow.SLINSF.SimulinkMan.removeBlockPreDeleteFcn  PreDeleteFcn=Stateflow.SLINSF.SimulinkMan.unsafePredeleteFcn
  Compare To Constant : simulink/Logic and Bit Operations/Compare To Constant  relop=>  const=RAMP_STEP_SIZE  OutDataTypeStr=boolean
  Constant : Constant  Value=0  OutDataTypeStr=Inherit: Inherit via back propagation
  Data Type Duplicate : DataTypeDuplicate
  Sum : Sum  Inputs=+-  RndMeth=Simplest  OutDataTypeStr=Inherit: Same as first input
  Switch : Switch  Criteria=u2 > Threshold  SaturateOnIntegerOverflow=off  InputSameDT=off
  Id0_out : Outport
  wires:
  Id0_in/1 -> Data Type Duplicate/1, Sum/1
  RAMP_STEP_SIZE/1 -> Sum/2
  Sum/1 -> Compare To Constant/1, Switch/1
  Compare To Constant/1 -> Switch/2
  Constant/1 -> Data Type Duplicate/2, Switch/3
  Switch/1 -> Id0_out/1

== system mcb_pmsm_foc_sensorless_f28069MLaunchPad/Current Control/Closed Loop/Current_Controllers ==
  Id : Inport
  Iq : Inport  Port=2
  Idq_Ref : Inport  Port=3
  DQ Limiter : mcbcontrolslib/DQ Limiter  satMethodInputType=Specify via dialog  satMethodSelected=D-Q equivalence  satLimitInputType=Specify via dialog  Vmax=1
  Demux : Demux  Outputs=2
  Mux : Mux
  PI_Controller_Id : Subsystem
  PI_Controller_Iq : Subsystem
  Terminator : Terminator
  Vd_ref : Outport  VectorParamsAs1DForOutWhenUnconnected=off
  Vq_ref : Outport  Port=2  VectorParamsAs1DForOutWhenUnconnected=off
  Idq : Outport  Port=3  VectorParamsAs1DForOutWhenUnconnected=off
  wires:
  Iq/1 -> Mux/4, PI_Controller_Iq/2(I_fb)  "Iq_fb"
  PI_Controller_Id/1(V_ref) -> DQ Limiter/1
  Id/1 -> PI_Controller_Id/2(I_fb), Mux/2  "Id_fb"
  Demux/1 -> PI_Controller_Id/1(I_ref), Mux/1  "Id_Ref"
  Demux/2 -> Mux/3, PI_Controller_Iq/1(I_ref)  "Iq_Ref"
  DQ Limiter/1 -> Vd_ref/1
  DQ Limiter/2 -> Vq_ref/1
  PI_Controller_Iq/1(V_ref) -> DQ Limiter/2
  DQ Limiter/3 -> Terminator/1
  Idq_Ref/1 -> Demux/1
  Mux/1 -> Idq/1

== system mcb_pmsm_foc_sensorless_f28069MLaunchPad/Current Control/Closed Loop/Open_Loop_Control ==
  Pos_PU : Inport
  Accumulate1 : Subsystem
      settings: LibrarySourceBlock=mcbcontrolslib/Position Generator/Accumulate
  Data Store Read : DataStoreRead  DataStoreName=SpdCtrlRef  IndexOptions=Index vector (dialog)  Indices=1  OutputSizes=1
  Data Store Read1 : DataStoreRead  DataStoreName=EnClosedLoop  IndexOptions=Index vector (dialog)  Indices=1  OutputSizes=1
  Data Store Read2 : DataStoreRead  DataStoreName=EnClosedLoop  IndexOptions=Index vector (dialog)  Indices=1  OutputSizes=1
  Delay : Delay  DelayLength=1  InitialConditionSource=Input port  ExternalReset=Falling
      settings: InputPortMap=u0,r5,p4
  Gain : Gain  Gain=Ts*PU_System.N_base*pmsm.p/60  OutDataTypeStr=Inherit: Same as input  ParamDataTypeStr=Inherit: Same as input
  Scope : Scope
  Switch : Switch  Criteria=u2 ~= 0  Threshold=0.1  SaturateOnIntegerOverflow=off  InputSameDT=off
  Pos_PU_Out : Outport
  wires:
  Pos_PU/1 -> Delay/3, Switch/1  "SMO_Pos"
  Switch/1 -> Pos_PU_Out/1
  Gain/1 -> Accumulate1/1(Theta)
  Data Store Read/1 -> Gain/1  "Spd_Pos"
  Data Store Read1/1 -> Switch/2
  Accumulate1/1(theta_e) -> Delay/1, Scope/1, Switch/3  "Pos_OL"
  Delay/1 -> Accumulate1/2(Theta_e_prev)
  Data Store Read2/1 -> Delay/2

== system mcb_pmsm_foc_sensorless_f28069MLaunchPad/Current Control/Data_Logging/Data ==
  Data : Inport
  Data_width : Inport  Port=2
  Action Port : ActionPort  ActionPortLabel=else
  Mux : Mux  Inputs=2
  Start : Constant  Value=hex2dec('0000')  OutDataTypeStr=uint16
  Data_out : Outport  VectorParamsAs1DForOutWhenUnconnected=off
  Iteration : Outport  Port=2  VectorParamsAs1DForOutWhenUnconnected=off
  wires:
  Start/1 -> Mux/2
  Mux/1 -> Data_out/1
  Data/1 -> Mux/1
  Data_width/1 -> Iteration/1

== system mcb_pmsm_foc_sensorless_f28069MLaunchPad/Current Control/Data_Logging/Data_Conditioning ==
  In1 : Inport
  Data Type Conversion : DataTypeConversion  OutDataTypeStr=fixdt(1,16,12)  RndMeth=Simplest  SaturateOnIntegerOverflow=off
  Data Type Conversion3 : DataTypeConversion  OutDataTypeStr=uint16  ConvertRealWorld=Stored Integer (SI)  SaturateOnIntegerOverflow=off  RndMeth=Floor
  Out1 : Outport  VectorParamsAs1DForOutWhenUnconnected=off
  wires:
  In1/1 -> Data Type Conversion/1
  Data Type Conversion3/1 -> Out1/1
  Data Type Conversion/1 -> Data Type Conversion3/1

== system mcb_pmsm_foc_sensorless_f28069MLaunchPad/Current Control/Data_Logging/End ==
  Data : Inport
  Data_width : Inport  Port=2
  Action Port : ActionPort  ActionPortLabel=elseif(u1 == 599)
  Bias : Bias  Bias=1  SaturateOnIntegerOverflow=off
  Mux : Mux  Inputs=2
  Start : Constant  Value=hex2dec('4545')  OutDataTypeStr=uint16
  Data_out : Outport  VectorParamsAs1DForOutWhenUnconnected=off
  Iteration : Outport  Port=2  VectorParamsAs1DForOutWhenUnconnected=off
  wires:
  Mux/1 -> Data_out/1
  Data_width/1 -> Bias/1
  Start/1 -> Mux/2
  Bias/1 -> Iteration/1
  Data/1 -> Mux/1

== system mcb_pmsm_foc_sensorless_f28069MLaunchPad/Current Control/Data_Logging/Start ==
  Data : Inport
  Data_width : Inport  Port=2
  Action Port : ActionPort  ActionPortLabel=if(u1 == 0)
  Bias : Bias  Bias=1  SaturateOnIntegerOverflow=off
  End : Constant  Value=hex2dec('5353')  OutDataTypeStr=uint16
  Mux : Mux  Inputs=2
  Data_out : Outport  VectorParamsAs1DForOutWhenUnconnected=off
  Iteration : Outport  Port=2  VectorParamsAs1DForOutWhenUnconnected=off
  wires:
  End/1 -> Mux/1
  Mux/1 -> Data_out/1
  Data_width/1 -> Bias/1
  Bias/1 -> Iteration/1
  Data/1 -> Mux/2

== system mcb_pmsm_foc_sensorless_f28069MLaunchPad/Current Control/HW Inputs/Sensor Driver Blocks (codegen) ==
  Sim : Inport
  IA/IB Measurement : c2802xlib/ADC  blkParamProc=C2000  ADCModule=1  samplingMode=Simultaneous sample mode  ADCResolution=12-bit (Single-ended input)  useSOC1=SOC0  useSOC2=SOC0_SOC1  SOCAcquisitionWindow=7  SOCTriggerSource=ePWM1_ADCSOCA  SOCInterruptTrigger=No ADCINT  Ts=-1  dType=uint16  postInterrupt=on  interruptSel=ADCINT1  ADCINTContinuous=on  endma=off  chdma=1  conv1=ADCINA0  conv2=ADCINA0 and ADCINB0  conv1_Type4=ADCIN0  conv2_Type4=ADCIN0 and ADCIN1
  Terminator : Terminator
  Iab_ADC : Outport
  wires:
  IA/IB Measurement/1 -> Iab_ADC/1
  Sim/1 -> Terminator/1

== system mcb_pmsm_foc_sensorless_f28069MLaunchPad/Current Control/HW Inputs/Sensor Driver Blocks (sim) ==
  Sim : Inport
  Iab_ADC : Outport
  wires:
  Sim/1 -> Iab_ADC/1

== system mcb_pmsm_foc_sensorless_f28069MLaunchPad/Current Control/Input Scaling/Calculate Phase Currents ==
  Iab_ADC : Inport
  Add : Sum  Inputs=-+
  Data Store Read : DataStoreRead  DataStoreName=IaOffset  IndexOptions=Index vector (dialog)  Indices=1  OutputSizes=1
  Data Store Read1 : DataStoreRead  DataStoreName=IbOffset  IndexOptions=Index vector (dialog)  Indices=1  OutputSizes=1
  Data Type Conversion : DataTypeConversion  OutDataTypeStr=int32  ConvertRealWorld=Stored Integer (SI)  SaturateOnIntegerOverflow=off  RndMeth=Floor
  Data Type Conversion1 : DataTypeConversion  OutDataTypeStr=dataType  SaturateOnIntegerOverflow=off  RndMeth=Floor
  Data Type Conversion3 : DataTypeConversion  OutDataTypeStr=fixdt(1,32,17)  ConvertRealWorld=Stored Integer (SI)  RndMeth=Simplest  SaturateOnIntegerOverflow=off
  Inverting / Non-inverting Current measurement amplifier : Gain  Gain=inverter.invertingAmp  RndMeth=Simplest  OutDataTypeStr=Inherit: Same as input
  Mux1 : Mux  Inputs=2
  Q17 per unit conversion : ArithShift  BitShiftNumber=-6
  Iab_meas_PU : Outport  VectorParamsAs1DForOutWhenUnconnected=off
  wires:
  Mux1/1 -> Add/1
  Data Type Conversion/1 -> Add/2
  Q17 per unit conversion/1 -> Data Type Conversion3/1
  Add/1 -> Q17 per unit conversion/1
  Data Type Conversion3/1 -> Data Type Conversion1/1
  Iab_ADC/1 -> Data Type Conversion/1
  Data Type Conversion1/1 -> Inverting / Non-inverting Current measurement amplifier/1
  Data Store Read1/1 -> Mux1/2
  Data Store Read/1 -> Mux1/1
  Inverting / Non-inverting Current measurement amplifier/1 -> Iab_meas_PU/1

== system mcb_pmsm_foc_sensorless_f28069MLaunchPad/Current Control/Input Scaling/Calculate position and speed ==
  VI_fb : Inport
  Demux : Demux  Outputs=2
  EstimatorSelector : Constant  OutDataTypeStr=uint32
  Extended EMF Observer : Subsystem
  Flux Observer : Subsystem
  Merge : Merge  Inputs=3
  Sliding Mode Observer : Subsystem
  Switch Case : SwitchCase  CaseConditions={0,1,2}  ShowDefaultCase=off
  Pos_PU : Outport
  speed_PU : Outport  Port=2
  wires:
  VI_fb/1 -> Extended EMF Observer/1(InputSignals), Flux Observer/1(InputSignals), Sliding Mode Observer/1(InputSignals)
  Demux/1 -> Pos_PU/1
  Demux/2 -> speed_PU/1
  EstimatorSelector/1 -> Switch Case/1
  Sliding Mode Observer/1(Position/Speed) -> Merge/1
  Flux Observer/1(Position/Speed) -> Merge/2
  Merge/1 -> Demux/1
  Switch Case/2 -> Flux Observer/Action
  Switch Case/1 -> Sliding Mode Observer/Action
  Extended EMF Observer/1(Position/Speed) -> Merge/3
  Switch Case/3 -> Extended EMF Observer/Action
